simulink model "RetroalimentacionNoLineal_v1"  (R2026b)
settings: Solver=VariableStepAuto
values from neighbouring files (symbols this model uses):
  g = 9.80665    [Pendulo_Invertido.m]
  Jp = m2*l*l + I    (= 0.024)    [Pendulo_Invertido.m]
  k = m2*l    (= 0.06)    [Pendulo_Invertido.m]
  M = m1+m2    (= 0.7)    [Pendulo_Invertido.m]
  Meq = M + Jm/(r*r)    (= 0.779)    [Pendulo_Invertido.m]
settings Model: Creator=fedeb  LastModifiedBy=fedeb

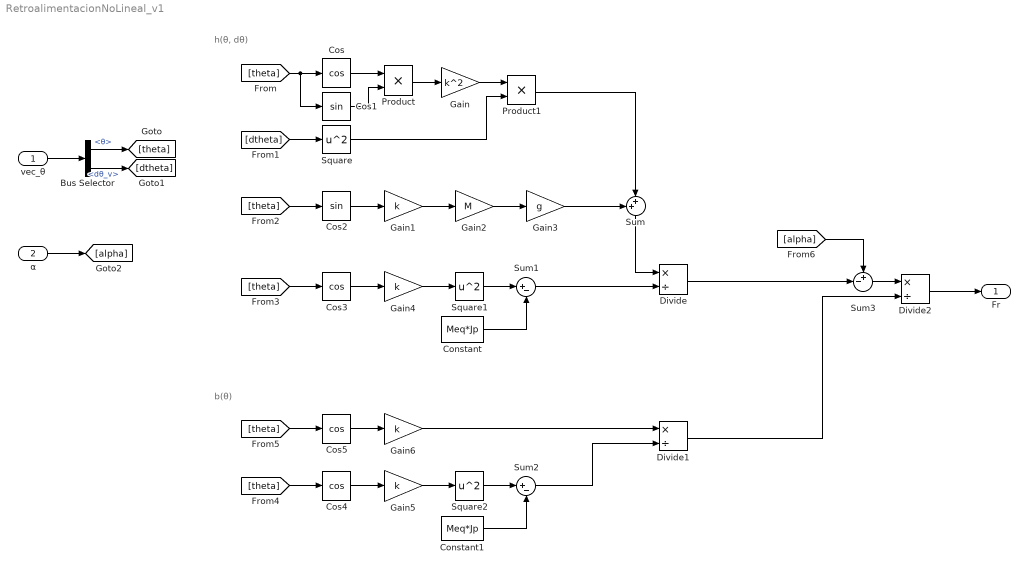
== system RetroalimentacionNoLineal_v1 ==
  note: b(θ)
  note: h(θ, dθ)
  vec_θ : Inport
  α : Inport  Port=2
  Bus Selector : BusSelector  OutputSignals=θ,dθ_v
  Constant : Constant  Value=Meq*Jp
  Constant1 : Constant  Value=Meq*Jp
  Cos{,3..5} (4 alike) : Trigonometry  Operator=cos
  Cos1 : Trigonometry
  Cos2 : Trigonometry
  Divide : Product  Inputs=*/
  Divide1 : Product  Inputs=*/
  Divide2 : Product  Inputs=*/
  Gain : Gain  Gain=k^2
  Gain{1,4..6} (4 alike) : Gain  Gain=k
  Gain2 : Gain  Gain=M
  Gain3 : Gain  Gain=g
  Product : Product
  Product1 : Product
  Square : Math  Operator=square
  Square1 : Math  Operator=square
  Square2 : Math  Operator=square
  Sum : Sum  Inputs=++|
  Sum1 : Sum  Inputs=|+-
  Sum2 : Sum  Inputs=|+-
  Sum3 : Sum  Inputs=+-|
  Fr : Outport
  wires:
  [theta] -> Cos/1, Cos1/1
  Product/1 -> Gain/1
  Cos/1 -> Product/1
  Cos1/1 -> Product/2
  Gain/1 -> Product1/1
  [dtheta] -> Square/1
  Square/1 -> Product1/2
  Product1/1 -> Sum/2
  [theta] -> Cos2/1
  Cos2/1 -> Gain1/1
  Gain1/1 -> Gain2/1
  Gain2/1 -> Gain3/1
  Gain3/1 -> Sum/1
  Sum/1 -> Divide/1
  [theta] -> Cos3/1
  Cos3/1 -> Gain4/1
  Sum1/1 -> Divide/2
  Gain4/1 -> Square1/1
  Square1/1 -> Sum1/1
  Gain5/1 -> Square2/1
  [theta] -> Cos4/1
  Square2/1 -> Sum2/1
  Gain6/1 -> Divide1/1
  Sum2/1 -> Divide1/2
  Cos4/1 -> Gain5/1
  Cos5/1 -> Gain6/1
  [theta] -> Cos5/1
  α/1 -> [alpha]
  [alpha] -> Sum3/1
  Divide/1 -> Sum3/2
  Sum3/1 -> Divide2/1
  Divide1/1 -> Divide2/2
  Divide2/1 -> Fr/1
  vec_θ/1 -> Bus Selector/1
  Bus Selector/1 -> [theta]  "<θ>"
  Bus Selector/2 -> [dtheta]  "<dθ_v>"
  Constant/1 -> Sum1/2
  Constant1/1 -> Sum2/2
